simulink model "MODELE"  (R2020a)
settings: Solver=ode23t  StartTime=0.0  StopTime=86400  RelTol=1e-3
libraries: fl_lib x11, nesl_utility x5, simulink x4
settings Model: Creator=dounia  LastModifiedBy=HP
settings SolverCC: ZeroCrossAlgorithm=Adaptive
settings DebuggingCC: IgnoredZcDiagnostic=none

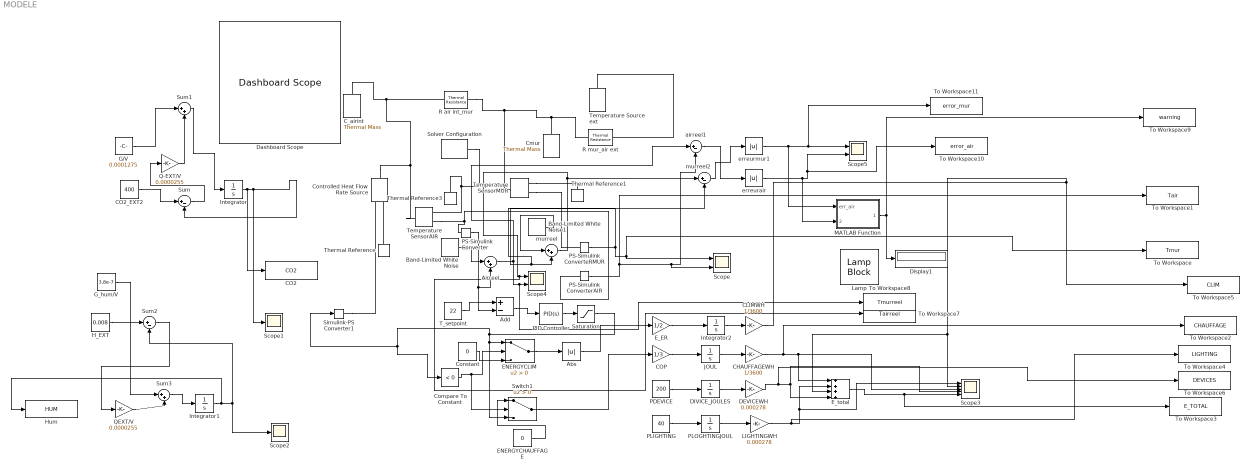
== system MODELE ==
  Abs : Abs
  Add : Sum  Inputs=+-
  Airreel : Sum  Inputs=|++
  Band-Limited White Noise : simulink/Sources/Band-Limited White Noise  Cov=0.02  Ts=0.1  seed=[23341]
  Band-Limited White Noise1 : simulink/Sources/Band-Limited White Noise  Cov=0.005  Ts=5  seed=[23341]
  CHAUFFAGEWH : Gain  Gain=1/3600
  CLIMWH : Gain  Gain=1/3600
  CO2 : ToWorkspace  VariableName=CO2  SaveFormat=Timeseries  SampleTime=-1
  CO2_EXT2 : Constant  Value=400
  COP : Gain  Gain=1/3
  C_airint : fl_lib/Thermal/Thermal Elements/Thermal Mass  mass=30 kg  sp_heat=1000 J/kg/K  T_specify=on  T_priority=High  T=20 degC  T_nominal_specify=off  T_nominal_unit=K  T_nominal_value=1  Q_specify=off  Q_priority=None  Q=0 W  Q_nominal_specify=off  Q_nominal_unit=W  Q_nominal_value=1
  Cmur : fl_lib/Thermal/Thermal Elements/Thermal Mass  mass=500 kg  sp_heat=5000 J/kg/K  T_specify=on  T_priority=High  T=25 degC  T_nominal_specify=off  T_nominal_unit=K  T_nominal_value=1  Q_specify=off  Q_priority=None  Q=0 W  Q_nominal_specify=off  Q_nominal_unit=W  Q_nominal_value=1
  Compare To Constant : simulink/Logic and Bit Operations/Compare To Constant  relop=<  const=0  OutDataTypeStr=boolean
  Constant : Constant  Value=0
  Controlled Heat Flow Rate Source : fl_lib/Thermal/Thermal Sources/Controlled Heat Flow Rate Source
  DEVICEWH : Gain  Gain=0.000278
  DIVICE_JOULES : Integrator
  Dashboard Scope : DashboardScope  TimeSpan=100  Ymin=15  Ymax=30
  Display1 : Display
  ENERGYCHAUFFAGE : Constant  Value=0
  ENERGYCLIM : Switch  Criteria=u2 > Threshold
  E_ER : Gain  Gain=1/2
  E_total : Sum  Inputs=++++
  G/V : Constant  Value=0.0001275
  G_hum/V : Constant  Value=3.8e-7
  H_EXT : Constant  Value=0.008
  Hum : ToWorkspace  VariableName=HUM  SaveFormat=Timeseries  SampleTime=-1
  Integrator : Integrator  InitialCondition=400
  Integrator1 : Integrator  InitialCondition=0.008
  Integrator2 : Integrator
  JOUL : Integrator
  LIGHTINGWH : Gain  Gain=0.000278
  Lamp : LampBlock
  MATLAB Function : MATLAB Function  TreatAsAtomicUnit=on
  PDEVICE : Constant  Value=200
  PID Controller : simulink/Continuous/PID Controller  Controller=PID  Form=Parallel  TimeDomain=Continuous-time  UseExternalTs=off  SampleTime=-1  IntegratorMethod=Forward Euler  FilterMethod=Forward Euler  ControllerParametersSource=internal  P=300  I=0.5  D=1  UseFilter=on  N=100  TunerSelectOption=Transfer Function Based (PID Tuner App)  InitialConditionSource=internal  InitialConditionForIntegrator=0  InitialConditionForFilter=0  DifferentiatorICPrevScaledInput=0  ExternalReset=none  TrackingMode=off  Kt=1  LimitOutput=on  UpperSaturationLimit=2000  LowerSaturationLimit=-2000  LinearizeAsGain=on  AntiWindupMode=none  Kb=1  POutMin=[]  POutMax=[]  IOutMin=[]  IOutMax=[]  DOutMin=[]  DOutMax=[]  NOutMin=[]  NOutMax=[]  SumOutMin=[]  SumOutMax=[]  SaturationOutMin=[]  SaturationOutMax=[]  PParamMin=[]  PParamMax=[]  IParamMin=[]  IParamMax=[]  DParamMin=[]  DParamMax=[]  NParamMin=[]  NParamMax=[]  KbParamMin=[]  KbParamMax=[]  KtParamMin=[]  KtParamMax=[]  KbOutMin=[]  KbOutMax=[]  KtOutMin=[]  KtOutMax=[]  IntegratorOutMin=[]  IntegratorOutMax=[]  FilterOutMin=[]  FilterOutMax=[]  SumI1OutMin=[]  SumI1OutMax=[]  SumI2OutMin=[]  SumI2OutMax=[]  SumI3OutMin=[]  SumI3OutMax=[]  SumI4OutMin=[]  SumI4OutMax=[]  SumDOutMin=[]  SumDOutMax=[]  DifferentiatorOutMin=[]  DifferentiatorOutMax=[]  FilterDiffOutCoefMin=[]  FilterDiffOutCoefMax=[]  ReciprocalOutMin=[]  ReciprocalOutMax=[]  SumDenOutMin=[]  SumDenOutMax=[]  SumNumOutMin=[]  SumNumOutMax=[]  DivideOutMin=[]  DivideOutMax=[]  UdiffTsProdOutMin=[]  UdiffTsProdOutMax=[]  NTsProdOutMin=[]  NTsProdOutMax=[]  UintegralTsProdOutMin=[]  UintegralTsProdOutMax=[]  UngainTsProdOutMin=[]  UngainTsProdOutMax=[]  IntegratorContinuousStateAttributes=''  IntegratorStateMustResolveToSignalObject=off  IntegratorRTWStateStorageClass=Auto  FilterContinuousStateAttributes=''  FilterStateMustResolveToSignalObject=off  FilterRTWStateStorageClass=Auto  ParallelPVariant=InternalParameters  IdealPVariant=Disabled  IVariant=InternalParameters  DVariant=InternalParameters  IntegratorVariant=Continuous  SatVariant=Enabled  AWVariant=Passthrough  PCopyVariant=Disabled  TRVariant=Disabled  FdbkBlocksVariant=Forward  IdealPFdbkVariant=Disabled  SatFdbkVariant=Disabled  DerivativeFilterVariant=ContFilter  NVariant=InternalParameters  NCopyVariant=Disabled  FilterICVariant=InternalICsFilter  IntegratorICVariant=InternalICs  ExternalResetVariant=Disabled  TRSumVariant=Passthrough  SumFdbkVariant=Disabled  SumVariant=Sum_PID  TsampFilterVariant=InternalTs  TsampNgainVariant=Passthrough  TsampIntegralVariant=Passthrough
  PLIGHTING : Constant  Value=40
  PLOGHTINGJOUL : Integrator
  PS-Simulink ConverteRMUR : nesl_utility/PS-Simulink Converter  PhysicalDomain=network_engine_domain  SubClassName=ps_output  LeftPortType=input  RightPortType=output  PseudoPeriodic=off  Frequencies=[]  Unit=degC  AffineConversion=on
  PS-Simulink Converter : nesl_utility/PS-Simulink Converter  PhysicalDomain=network_engine_domain  SubClassName=ps_output  LeftPortType=input  RightPortType=output  PseudoPeriodic=off  Frequencies=[]  Unit=degC  AffineConversion=on
  PS-Simulink ConverterAIR : nesl_utility/PS-Simulink Converter  PhysicalDomain=network_engine_domain  SubClassName=ps_output  LeftPortType=input  RightPortType=output  PseudoPeriodic=off  Frequencies=[]  Unit=degC  AffineConversion=on
  Q-EXT/V : Gain  Gain=0.0000255
  QEXT/V : Gain  Gain=0.0000255
  R air int_mur : fl_lib/Thermal/Thermal Elements/Thermal Resistance  resistance=0.5 K/W  T_specify=off  T_priority=None  T=0 K  T_nominal_specify=off  T_nominal_unit=K  T_nominal_value=1  Q_specify=off  Q_priority=None  Q=0 W  Q_nominal_specify=off  Q_nominal_unit=W  Q_nominal_value=1
      settings: SourceProductBaseCode=SS
  R mur_air ext : fl_lib/Thermal/Thermal Elements/Thermal Resistance  resistance=2 K/W  T_specify=off  T_priority=None  T=0 K  T_nominal_specify=off  T_nominal_unit=K  T_nominal_value=1  Q_specify=off  Q_priority=None  Q=0 W  Q_nominal_specify=off  Q_nominal_unit=W  Q_nominal_value=1
      settings: SourceProductBaseCode=SS
  Saturation : Saturate  UpperLimit=2000  LowerLimit=-2000
  Scope : Scope  NumInputPorts=2
  Scope1 : Scope
  Scope2 : Scope
  Scope3 : Scope  NumInputPorts=5
  Scope4 : Scope  NumInputPorts=2
  Scope5 : Scope  NumInputPorts=2
  Simulink-PS Converter1 : nesl_utility/Simulink-PS Converter  PhysicalDomain=network_engine_domain  SubClassName=ps_input  LeftPortType=input  RightPortType=output  PseudoPeriodic=off  Frequencies=[]  NoiseDistribution=none  NoiseParameters=[]  Unit=W  AffineConversion=on  FilteringAndDerivatives=provide  SimscapeFilterOrder=1  InputFilterTimeConstant=0.001  UdotUserProvided=0
  Solver Configuration : nesl_utility/Solver Configuration  PhysicalDomain=network_engine_domain  SubClassName=solver  LeftPortType=input  RightPortType=generic  Tones=[]  Harmonics=[]  SimulateNoise=off  Profile=off  UseLocalSampling=off  EnableSwitchedLinearOptims=on  FrequencyDomain=off  UseCCode=off  RelTol=0.001  AbsTol=1e-06  MinStep=1e-09  ToWorkspace=off  RevertToSquareIcSolve=off  NumHomotopyIterations=100  PhasorMode=off  PhasorModeNumHarmonics=1  DoDC=off  ResidualTolerance=1e-09  UseLocalSolver=off  LocalSolverChoice=NE_BACKWARD_EULER_ADVANCER  LocalSolverSampleTime=0.001  DoFixedCost=off  MaxNonlinIter=3  MaxModeIter=2  LinearAlgebra=auto  EquationFormulation=NE_TIME_EF  DelaysMemoryBudget=1024  AutomaticFiltering=on  FilteringTimeConstant=0.001  PartitionStorageMethod=AS_NEEDED  PartitionMemoryBudget=1024  PartitionMethod=ROBUST
  Sum : Sum  Inputs=|+-
  Sum1 : Sum  Inputs=|++
  Sum2 : Sum  Inputs=|+-
  Sum3 : Sum  Inputs=|++
  Switch1 : Switch  Criteria=u2 > Threshold
  T_setpoint : Constant  Value=22
  Temperature SensorAIR : fl_lib/Thermal/Thermal Sensors/Temperature Sensor
  Temperature SensorMUR : fl_lib/Thermal/Thermal Sensors/Temperature Sensor
  Temperature Source ext : fl_lib/Thermal/Thermal Sources/Temperature Source  temperature=30 degC
  Thermal Reference : fl_lib/Thermal/Thermal Elements/Thermal Reference
  Thermal Reference1 : fl_lib/Thermal/Thermal Elements/Thermal Reference
  Thermal Reference3 : fl_lib/Thermal/Thermal Elements/Thermal Reference
  To Workspace : ToWorkspace  VariableName=Tmur  SaveFormat=Timeseries  SampleTime=-1
  To Workspace1 : ToWorkspace  VariableName=Tair  SaveFormat=Timeseries  SampleTime=-1
  To Workspace10 : ToWorkspace  VariableName=error_air  SaveFormat=Timeseries  SampleTime=-1
  To Workspace11 : ToWorkspace  VariableName=error_mur  SaveFormat=Timeseries  SampleTime=-1
  To Workspace2 : ToWorkspace  VariableName=CHAUFFAGE  SaveFormat=Timeseries  SampleTime=-1
  To Workspace3 : ToWorkspace  VariableName=E_TOTAL  SaveFormat=Timeseries  SampleTime=-1
  To Workspace4 : ToWorkspace  VariableName=LIGHTING  SaveFormat=Timeseries  SampleTime=-1
  To Workspace5 : ToWorkspace  VariableName=CLIM  SaveFormat=Timeseries  SampleTime=-1
  To Workspace6 : ToWorkspace  VariableName=DEVICES  SaveFormat=Timeseries  SampleTime=-1
  To Workspace7 : ToWorkspace  VariableName=Tairreel  SaveFormat=Timeseries  SampleTime=-1
  To Workspace8 : ToWorkspace  VariableName=Tmurreel  SaveFormat=Timeseries  SampleTime=-1
  To Workspace9 : ToWorkspace  VariableName=warning  SaveFormat=Timeseries  SampleTime=-1
  airreel1 : Sum  Inputs=|+-
  erreurair : Abs
  erreurmur1 : Abs
  murreel : Sum  Inputs=|++
  murreel2 : Sum  Inputs=|+-
  wires:
  PS-Simulink ConverteRMUR/1 -> murreel/2, murreel2/2, To Workspace/1, Scope/1
  PS-Simulink ConverterAIR/1 -> To Workspace1/1, airreel1/2, Scope/2
  COP/1 -> JOUL/1
  JOUL/1 -> CHAUFFAGEWH/1
  PLIGHTING/1 -> PLOGHTINGJOUL/1
  PLOGHTINGJOUL/1 -> LIGHTINGWH/1
  PDEVICE/1 -> DIVICE_JOULES/1
  DIVICE_JOULES/1 -> DEVICEWH/1
  CHAUFFAGEWH/1 -> To Workspace2/1, Scope3/3, E_total/1
  DEVICEWH/1 -> To Workspace6/1, Scope3/4, E_total/4
  LIGHTINGWH/1 -> To Workspace4/1, Scope3/1, E_total/2
  E_total/1 -> To Workspace3/1, Scope3/5
  CO2_EXT2/1 -> Sum/1
  G/V/1 -> Sum1/1
  Q-EXT/V/1 -> Sum1/2
  Sum1/1 -> Integrator/1
  Sum/1 -> Q-EXT/V/1
  Integrator/1 -> CO2/1, Sum/2, Scope1/1
  G_hum/V/1 -> Sum3/1
  Sum3/1 -> Integrator1/1
  H_EXT/1 -> Sum2/1
  Sum2/1 -> QEXT/V/1
  QEXT/V/1 -> Sum3/2
  Integrator1/1 -> Hum/1, Scope2/1, Sum2/2
  T_setpoint/1 -> Add/1
  Add/1 -> PID Controller/1
  PS-Simulink Converter/1 -> Add/2, Airreel/2
  PID Controller/1 -> Saturation/1
  Saturation/1 -> Compare To Constant/1, Simulink-PS Converter1/1, Switch1/3, ENERGYCLIM/1
  Switch1/1 -> COP/1
  Compare To Constant/1 -> Switch1/2, ENERGYCLIM/2
  Constant/1 -> ENERGYCLIM/3
  ENERGYCHAUFFAGE/1 -> Switch1/1
  ENERGYCLIM/1 -> Abs/1
  Abs/1 -> E_ER/1
  E_ER/1 -> Integrator2/1
  Integrator2/1 -> CLIMWH/1
  CLIMWH/1 -> E_total/3, Scope3/2, To Workspace5/1
  Band-Limited White Noise/1 -> Airreel/1
  Airreel/1 -> To Workspace8/1, Scope4/2, airreel1/1
  Band-Limited White Noise1/1 -> murreel/1
  murreel/1 -> murreel2/1, To Workspace7/1, Scope4/1
  airreel1/1 -> erreurair/1
  erreurair/1 -> MATLAB Function/2(err_mur), To Workspace10/1, Scope5/2
  murreel2/1 -> erreurmur1/1
  erreurmur1/1 -> MATLAB Function/1(err_air), To Workspace11/1, Scope5/1
  MATLAB Function/1(warning) -> Display1/1, To Workspace9/1
  connections:
  Controlled Heat Flow Rate Source/LConn1 -- C_airint/LConn1 -- R air int_mur/LConn1 -- Temperature SensorAIR/LConn1
  R air int_mur/RConn1 -- Temperature SensorMUR/LConn1 -- R mur_air ext/LConn1 -- Cmur/LConn1
  Thermal Reference/LConn1 -- Controlled Heat Flow Rate Source/RConn2
  Temperature SensorAIR/RConn2 -- PS-Simulink Converter/LConn1 -- PS-Simulink ConverterAIR/LConn1
  Temperature SensorMUR/RConn1 -- Thermal Reference1/LConn1
  Temperature SensorMUR/RConn2 -- PS-Simulink ConverteRMUR/LConn1
  Solver Configuration/RConn1 -- Temperature SensorAIR/RConn1 -- Thermal Reference3/LConn1
  Simulink-PS Converter1/RConn1 -- Controlled Heat Flow Rate Source/RConn1
  Temperature Source ext/LConn1 -- R mur_air ext/RConn1

== matlab function MODELE/MATLAB Function ==
  data: err_air input; err_mur input; warning output
function warning = warning_signal(err_air, err_mur)

if err_air > 0.5 || err_mur > 0.5
    warning = 1;
else
    warning = 0;
end
